simulink model "OpenXstim_Stage2A_Linear"  (R2025a)
settings: Solver=FixedStepDiscrete  StartTime=0  StopTime=60  FixedStep=0.082500000000000004  RelTol=1e-3
settings Model: Creator=arnav  LastModifiedBy=arnav

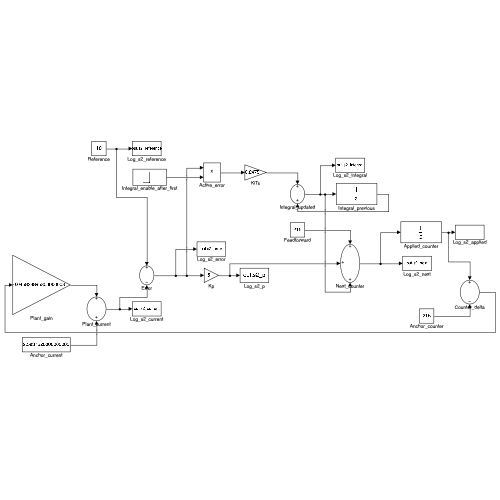
[thumbnail: Simulink's stored preview of the top-level diagram]
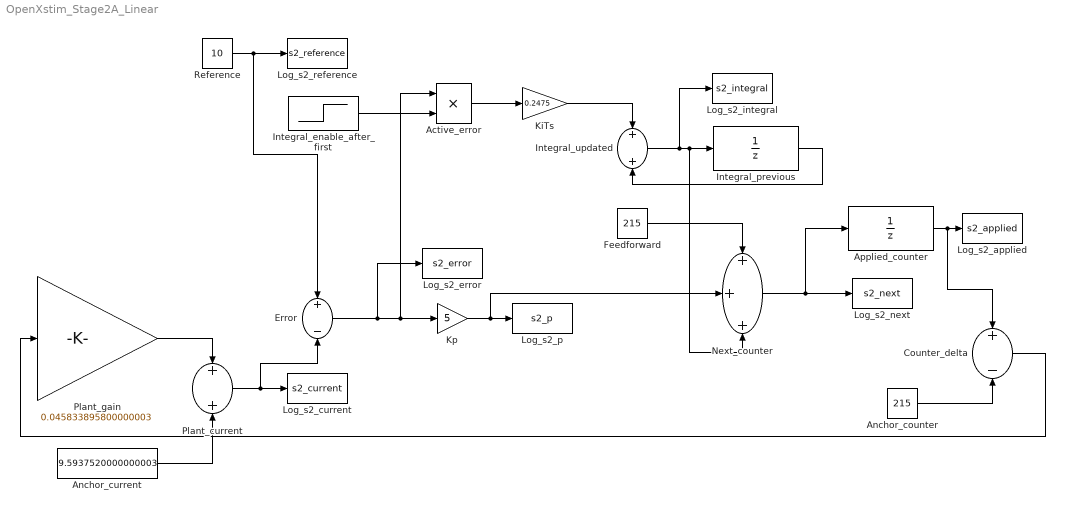
== system OpenXstim_Stage2A_Linear ==
  Active_error : Product
  Anchor_counter : Constant  Value=215
  Anchor_current : Constant  Value=9.5937520000000003
  Applied_counter : UnitDelay  InitialCondition=215  SampleTime=0.082500000000000004  HasFrameUpgradeWarning=on
  Counter_delta : Sum  Inputs=+-
  Error : Sum  Inputs=+-
  Feedforward : Constant  Value=215
  Integral_enable_after_first : Step  Time=0.041250000000000002  SampleTime=0.082500000000000004
  Integral_previous : UnitDelay  SampleTime=0.082500000000000004  HasFrameUpgradeWarning=on
  Integral_updated : Sum
  KiTs : Gain  Gain=0.2475
  Kp : Gain  Gain=5
  Log_s2_applied : ToWorkspace  VariableName=s2_applied  SaveFormat=Timeseries  SampleTime=-1
  Log_s2_current : ToWorkspace  VariableName=s2_current  SaveFormat=Timeseries  SampleTime=-1
  Log_s2_error : ToWorkspace  VariableName=s2_error  SaveFormat=Timeseries  SampleTime=-1
  Log_s2_integral : ToWorkspace  VariableName=s2_integral  SaveFormat=Timeseries  SampleTime=-1
  Log_s2_next : ToWorkspace  VariableName=s2_next  SaveFormat=Timeseries  SampleTime=-1
  Log_s2_p : ToWorkspace  VariableName=s2_p  SaveFormat=Timeseries  SampleTime=-1
  Log_s2_reference : ToWorkspace  VariableName=s2_reference  SaveFormat=Timeseries  SampleTime=-1
  Next_counter : Sum  Inputs=+++
  Plant_current : Sum
  Plant_gain : Gain  Gain=0.045833895800000003
  Reference : Constant  Value=10
  wires:
  Next_counter/1 -> Log_s2_next/1, Applied_counter/1
  Plant_current/1 -> Log_s2_current/1, Error/2
  Feedforward/1 -> Next_counter/1
  Anchor_counter/1 -> Counter_delta/2
  Integral_updated/1 -> Integral_previous/1, Next_counter/3, Log_s2_integral/1
  Active_error/1 -> KiTs/1
  Counter_delta/1 -> Plant_gain/1
  Kp/1 -> Log_s2_p/1, Next_counter/2
  Anchor_current/1 -> Plant_current/2
  KiTs/1 -> Integral_updated/1
  Integral_enable_after_first/1 -> Active_error/2
  Integral_previous/1 -> Integral_updated/2
  Reference/1 -> Log_s2_reference/1, Error/1
  Applied_counter/1 -> Log_s2_applied/1, Counter_delta/1
  Error/1 -> Kp/1, Active_error/1, Log_s2_error/1
  Plant_gain/1 -> Plant_current/1
